simulink model "Link_MCU_GNC"  (R2026b)
settings: Solver=VariableStepAuto
undefined symbols (not defined in the file or in its folder): P, Ts
settings Model: Creator=aomar  LastModifiedBy=aomar

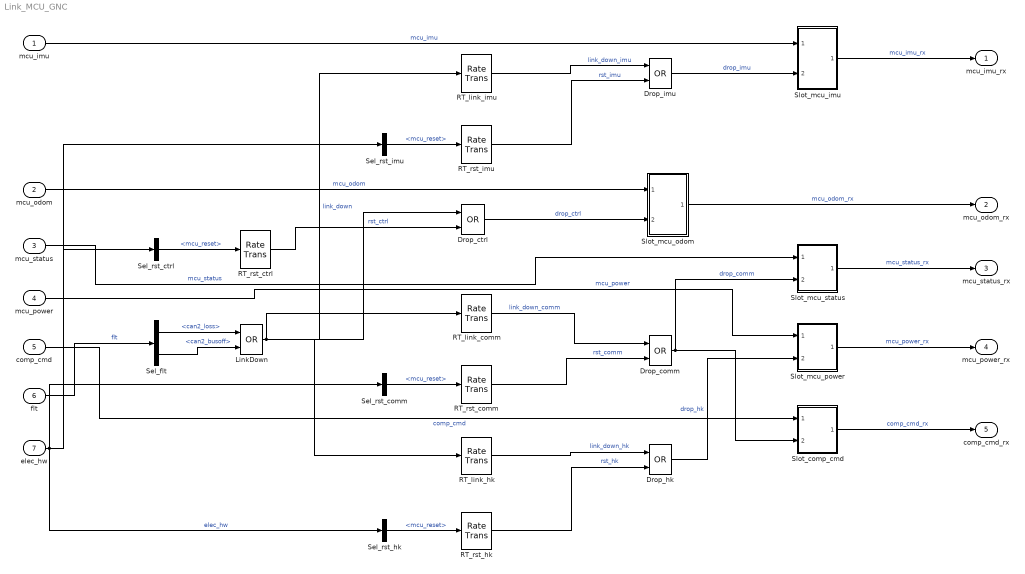
== system Link_MCU_GNC ==
  mcu_imu : Inport  OutDataTypeStr=Bus: Bus_CanFrame64  SampleTime=Ts.imu
  mcu_odom : Inport  Port=2  OutDataTypeStr=Bus: Bus_CanFrame64  SampleTime=Ts.ctrl
  mcu_status : Inport  Port=3  OutDataTypeStr=Bus: Bus_CanFrame64  SampleTime=Ts.comm
  mcu_power : Inport  Port=4  OutDataTypeStr=Bus: Bus_CanFrame64  SampleTime=Ts.hk
  comp_cmd : Inport  Port=5  OutDataTypeStr=Bus: Bus_CanFrame64  SampleTime=Ts.comm
  flt : Inport  Port=6  OutDataTypeStr=Bus: Bus_FaultInject  SampleTime=Ts.ctrl
  elec_hw : Inport  Port=7  OutDataTypeStr=Bus: Bus_ElecHwIn  SampleTime=Ts.base
  Drop_comm : Logic  Operator=OR  AllPortsSameDT=off  OutDataTypeStr=boolean
  Drop_ctrl : Logic  Operator=OR  AllPortsSameDT=off  OutDataTypeStr=boolean
  Drop_hk : Logic  Operator=OR  AllPortsSameDT=off  OutDataTypeStr=boolean
  Drop_imu : Logic  Operator=OR  AllPortsSameDT=off  OutDataTypeStr=boolean
  LinkDown : Logic  Operator=OR  AllPortsSameDT=off  OutDataTypeStr=boolean
  RT_link_comm : RateTransition  InitialCondition=false  OutPortSampleTime=Ts.comm
  RT_link_hk : RateTransition  InitialCondition=false  OutPortSampleTime=Ts.hk
  RT_link_imu : RateTransition  InitialCondition=false  OutPortSampleTime=Ts.imu
  RT_rst_comm : RateTransition  InitialCondition=false  OutPortSampleTime=Ts.comm
  RT_rst_ctrl : RateTransition  InitialCondition=false  OutPortSampleTime=Ts.ctrl
  RT_rst_hk : RateTransition  InitialCondition=false  OutPortSampleTime=Ts.hk
  RT_rst_imu : RateTransition  InitialCondition=false  OutPortSampleTime=Ts.imu
  Sel_flt : BusSelector  OutputSignals=can2_loss,can2_busoff
  Sel_rst_comm : BusSelector  OutputSignals=mcu_reset
  Sel_rst_ctrl : BusSelector  OutputSignals=mcu_reset
  Sel_rst_hk : BusSelector  OutputSignals=mcu_reset
  Sel_rst_imu : BusSelector  OutputSignals=mcu_reset
  Slot_comp_cmd : Subsystem
  Slot_mcu_imu : Subsystem
  Slot_mcu_odom : Subsystem
  Slot_mcu_power : Subsystem
  Slot_mcu_status : Subsystem
  mcu_imu_rx : Outport  OutDataTypeStr=Bus: Bus_CanFrame64
  mcu_odom_rx : Outport  Port=2  OutDataTypeStr=Bus: Bus_CanFrame64
  mcu_status_rx : Outport  Port=3  OutDataTypeStr=Bus: Bus_CanFrame64
  mcu_power_rx : Outport  Port=4  OutDataTypeStr=Bus: Bus_CanFrame64
  comp_cmd_rx : Outport  Port=5  OutDataTypeStr=Bus: Bus_CanFrame64
  wires:
  mcu_imu/1 -> Slot_mcu_imu/1(frame)  "mcu_imu"
  mcu_odom/1 -> Slot_mcu_odom/1(frame)  "mcu_odom"
  mcu_status/1 -> Slot_mcu_status/1(frame)  "mcu_status"
  mcu_power/1 -> Slot_mcu_power/1(frame)  "mcu_power"
  comp_cmd/1 -> Slot_comp_cmd/1(frame)  "comp_cmd"
  flt/1 -> Sel_flt/1  "flt"
  elec_hw/1 -> Sel_rst_imu/1, Sel_rst_ctrl/1, Sel_rst_hk/1, Sel_rst_comm/1  "elec_hw"
  Sel_rst_ctrl/1 -> RT_rst_ctrl/1  "<mcu_reset>"
  Sel_flt/1 -> LinkDown/1  "<can2_loss>"
  Sel_flt/2 -> LinkDown/2  "<can2_busoff>"
  LinkDown/1 -> RT_link_imu/1, Drop_ctrl/1, RT_link_hk/1, RT_link_comm/1  "link_down"
  RT_rst_ctrl/1 -> Drop_ctrl/2  "rst_ctrl"
  Sel_rst_imu/1 -> RT_rst_imu/1  "<mcu_reset>"
  Sel_rst_comm/1 -> RT_rst_comm/1  "<mcu_reset>"
  Sel_rst_hk/1 -> RT_rst_hk/1  "<mcu_reset>"
  Drop_ctrl/1 -> Slot_mcu_odom/2(drop)  "drop_ctrl"
  RT_link_imu/1 -> Drop_imu/1  "link_down_imu"
  RT_rst_imu/1 -> Drop_imu/2  "rst_imu"
  RT_link_comm/1 -> Drop_comm/1  "link_down_comm"
  RT_rst_comm/1 -> Drop_comm/2  "rst_comm"
  RT_link_hk/1 -> Drop_hk/1  "link_down_hk"
  RT_rst_hk/1 -> Drop_hk/2  "rst_hk"
  Drop_imu/1 -> Slot_mcu_imu/2(drop)  "drop_imu"
  Drop_comm/1 -> Slot_comp_cmd/2(drop), Slot_mcu_status/2(drop)  "drop_comm"
  Drop_hk/1 -> Slot_mcu_power/2(drop)  "drop_hk"
  Slot_mcu_odom/1(frame_rx) -> mcu_odom_rx/1  "mcu_odom_rx"
  Slot_mcu_imu/1(frame_rx) -> mcu_imu_rx/1  "mcu_imu_rx"
  Slot_mcu_status/1(frame_rx) -> mcu_status_rx/1  "mcu_status_rx"
  Slot_mcu_power/1(frame_rx) -> mcu_power_rx/1  "mcu_power_rx"
  Slot_comp_cmd/1(frame_rx) -> comp_cmd_rx/1  "comp_cmd_rx"

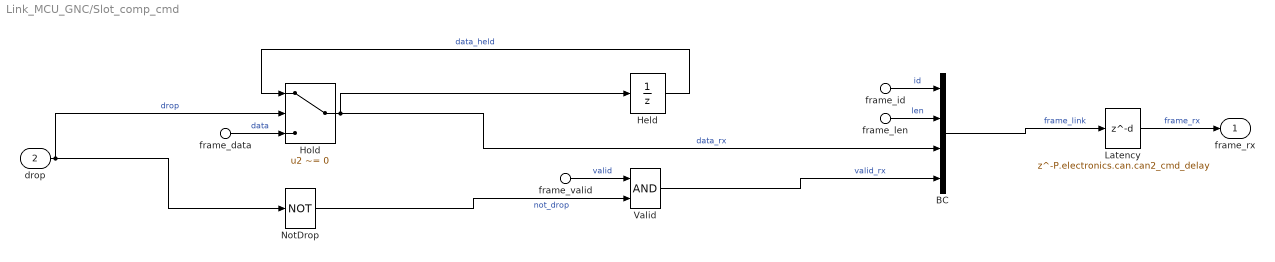
== system Link_MCU_GNC/Slot_comp_cmd ==
  frame_id : Inport  PortName=frame  Element=id
  frame_len : Inport  PortName=frame  Element=len
  frame_data : Inport  PortName=frame  Element=data
  frame_valid : Inport  PortName=frame  Element=valid
  drop : Inport  Port=2
  BC : BusCreator  Inputs=4  OutDataTypeStr=Bus: Bus_CanFrame64  NonVirtualBus=on
      settings: InheritFromInputs=off
  Held : UnitDelay  SampleTime=Ts.comm
  Hold : Switch  Criteria=u2 ~= 0  SaturateOnIntegerOverflow=off  InputSameDT=off
  Latency : Delay  DelayLength=P.electronics.can.can2_cmd_delay  InitialCondition=P.ic.Bus_CanFrame64  SampleTime=Ts.comm
  NotDrop : Logic  Operator=NOT  Inputs=1  AllPortsSameDT=off  OutDataTypeStr=boolean
  Valid : Logic  AllPortsSameDT=off  OutDataTypeStr=boolean
  frame_rx : Outport
  wires:
  drop/1 -> NotDrop/1, Hold/2  "drop"
  frame_data/1 -> Hold/3  "data"
  NotDrop/1 -> Valid/2  "not_drop"
  Hold/1 -> BC/3, Held/1  "data_rx"
  frame_valid/1 -> Valid/1  "valid"
  Valid/1 -> BC/4  "valid_rx"
  Held/1 -> Hold/1  "data_held"
  frame_id/1 -> BC/1  "id"
  frame_len/1 -> BC/2  "len"
  BC/1 -> Latency/1  "frame_link"
  Latency/1 -> frame_rx/1  "frame_rx"

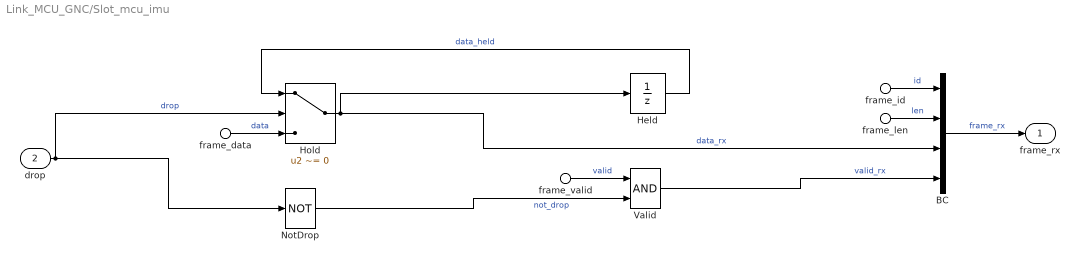
== system Link_MCU_GNC/Slot_mcu_imu ==
  frame_id : Inport  PortName=frame  Element=id
  frame_len : Inport  PortName=frame  Element=len
  frame_data : Inport  PortName=frame  Element=data
  frame_valid : Inport  PortName=frame  Element=valid
  drop : Inport  Port=2
  BC : BusCreator  Inputs=4  OutDataTypeStr=Bus: Bus_CanFrame64  NonVirtualBus=on
      settings: InheritFromInputs=off
  Held : UnitDelay  SampleTime=Ts.imu
  Hold : Switch  Criteria=u2 ~= 0  SaturateOnIntegerOverflow=off  InputSameDT=off
  NotDrop : Logic  Operator=NOT  Inputs=1  AllPortsSameDT=off  OutDataTypeStr=boolean
  Valid : Logic  AllPortsSameDT=off  OutDataTypeStr=boolean
  frame_rx : Outport
  wires:
  drop/1 -> NotDrop/1, Hold/2  "drop"
  frame_data/1 -> Hold/3  "data"
  NotDrop/1 -> Valid/2  "not_drop"
  Hold/1 -> BC/3, Held/1  "data_rx"
  frame_valid/1 -> Valid/1  "valid"
  Valid/1 -> BC/4  "valid_rx"
  Held/1 -> Hold/1  "data_held"
  frame_id/1 -> BC/1  "id"
  frame_len/1 -> BC/2  "len"
  BC/1 -> frame_rx/1  "frame_rx"

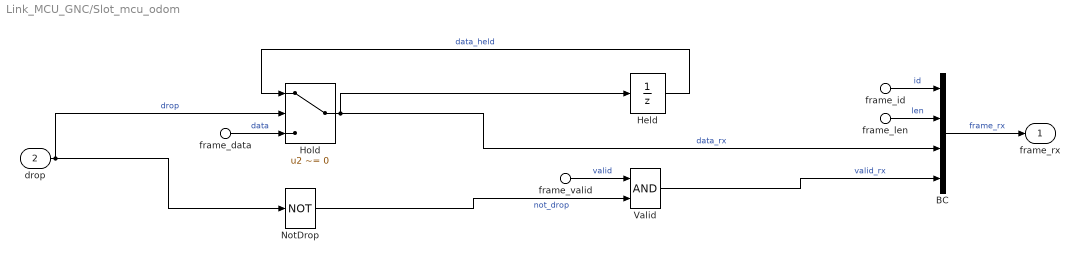
== system Link_MCU_GNC/Slot_mcu_odom ==
  frame_id : Inport  PortName=frame  Element=id
  frame_len : Inport  PortName=frame  Element=len
  frame_data : Inport  PortName=frame  Element=data
  frame_valid : Inport  PortName=frame  Element=valid
  drop : Inport  Port=2
  BC : BusCreator  Inputs=4  OutDataTypeStr=Bus: Bus_CanFrame64  NonVirtualBus=on
      settings: InheritFromInputs=off
  Held : UnitDelay  SampleTime=Ts.ctrl
  Hold : Switch  Criteria=u2 ~= 0  SaturateOnIntegerOverflow=off  InputSameDT=off
  NotDrop : Logic  Operator=NOT  Inputs=1  AllPortsSameDT=off  OutDataTypeStr=boolean
  Valid : Logic  AllPortsSameDT=off  OutDataTypeStr=boolean
  frame_rx : Outport
  wires:
  drop/1 -> NotDrop/1, Hold/2  "drop"
  frame_data/1 -> Hold/3  "data"
  NotDrop/1 -> Valid/2  "not_drop"
  Hold/1 -> BC/3, Held/1  "data_rx"
  frame_valid/1 -> Valid/1  "valid"
  Valid/1 -> BC/4  "valid_rx"
  Held/1 -> Hold/1  "data_held"
  frame_id/1 -> BC/1  "id"
  frame_len/1 -> BC/2  "len"
  BC/1 -> frame_rx/1  "frame_rx"

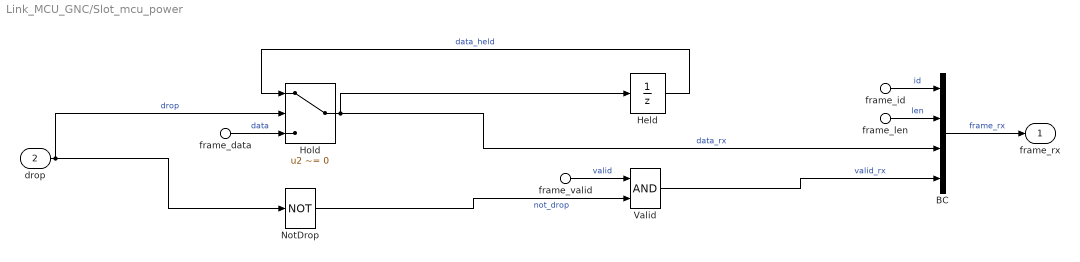
== system Link_MCU_GNC/Slot_mcu_power ==
  frame_id : Inport  PortName=frame  Element=id
  frame_len : Inport  PortName=frame  Element=len
  frame_data : Inport  PortName=frame  Element=data
  frame_valid : Inport  PortName=frame  Element=valid
  drop : Inport  Port=2
  BC : BusCreator  Inputs=4  OutDataTypeStr=Bus: Bus_CanFrame64  NonVirtualBus=on
      settings: InheritFromInputs=off
  Held : UnitDelay  SampleTime=Ts.hk
  Hold : Switch  Criteria=u2 ~= 0  SaturateOnIntegerOverflow=off  InputSameDT=off
  NotDrop : Logic  Operator=NOT  Inputs=1  AllPortsSameDT=off  OutDataTypeStr=boolean
  Valid : Logic  AllPortsSameDT=off  OutDataTypeStr=boolean
  frame_rx : Outport
  wires:
  drop/1 -> NotDrop/1, Hold/2  "drop"
  frame_data/1 -> Hold/3  "data"
  NotDrop/1 -> Valid/2  "not_drop"
  Hold/1 -> BC/3, Held/1  "data_rx"
  frame_valid/1 -> Valid/1  "valid"
  Valid/1 -> BC/4  "valid_rx"
  Held/1 -> Hold/1  "data_held"
  frame_id/1 -> BC/1  "id"
  frame_len/1 -> BC/2  "len"
  BC/1 -> frame_rx/1  "frame_rx"

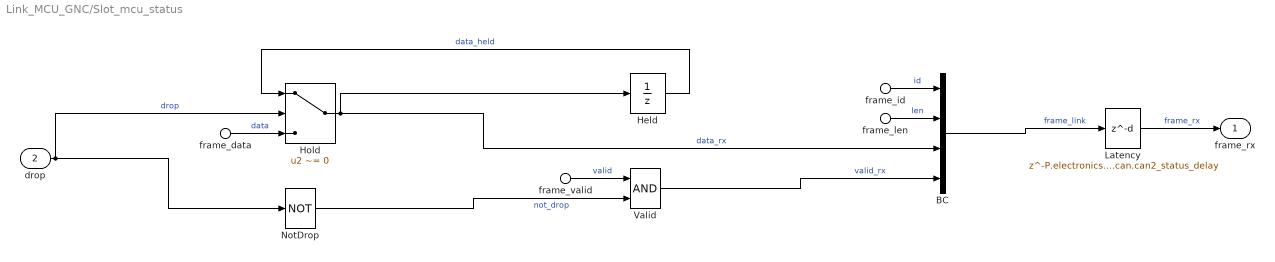
== system Link_MCU_GNC/Slot_mcu_status ==
  frame_id : Inport  PortName=frame  Element=id
  frame_len : Inport  PortName=frame  Element=len
  frame_data : Inport  PortName=frame  Element=data
  frame_valid : Inport  PortName=frame  Element=valid
  drop : Inport  Port=2
  BC : BusCreator  Inputs=4  OutDataTypeStr=Bus: Bus_CanFrame64  NonVirtualBus=on
      settings: InheritFromInputs=off
  Held : UnitDelay  SampleTime=Ts.comm
  Hold : Switch  Criteria=u2 ~= 0  SaturateOnIntegerOverflow=off  InputSameDT=off
  Latency : Delay  DelayLength=P.electronics.can.can2_status_delay  InitialCondition=P.ic.Bus_CanFrame64  PreventDirectFeedthrough=on  SampleTime=Ts.comm
  NotDrop : Logic  Operator=NOT  Inputs=1  AllPortsSameDT=off  OutDataTypeStr=boolean
  Valid : Logic  AllPortsSameDT=off  OutDataTypeStr=boolean
  frame_rx : Outport
  wires:
  drop/1 -> NotDrop/1, Hold/2  "drop"
  frame_data/1 -> Hold/3  "data"
  NotDrop/1 -> Valid/2  "not_drop"
  Hold/1 -> BC/3, Held/1  "data_rx"
  frame_valid/1 -> Valid/1  "valid"
  Valid/1 -> BC/4  "valid_rx"
  Held/1 -> Hold/1  "data_held"
  frame_id/1 -> BC/1  "id"
  frame_len/1 -> BC/2  "len"
  BC/1 -> Latency/1  "frame_link"
  Latency/1 -> frame_rx/1  "frame_rx"
